simulink model "tb_mcu_rc"  (R2026b)
values from neighbouring files (symbols this model uses):
  P = evalin('base', 'P')    [elec_harness.m]    (also in mcu_can1_roundtrip.m; mcu_can2_roundtrip.m; mcu_cl_input.m; mcu_ctrl_harness.m)
  Ts = prm(1)    [mcu_cl_track_dyn.m]    (also in mcu_ctrl_harness.m = evalin('base', tsExpr))
libraries: simulink x3
settings Model: Creator=aomar  LastModifiedBy=aomar

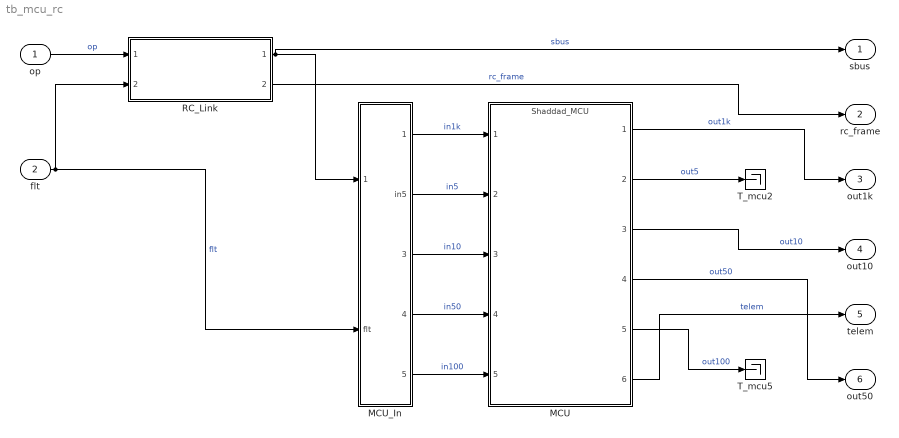
== system tb_mcu_rc ==
  op : Inport  OutDataTypeStr=Bus: Bus_OperatorCmd  SampleTime=Ts.ctrl
  flt : Inport  Port=2  OutDataTypeStr=Bus: Bus_FaultInject  SampleTime=Ts.ctrl
  MCU : ModelReference  ModelNameDialog=Shaddad_MCU  SimulationMode=Normal  ModelReferenceVersion=1.1
  MCU_In : Subsystem
  RC_Link : Subsystem  ReferencedSubsystem=RC_Link_Sim
  T_mcu2 : Terminator
  T_mcu5 : Terminator
  sbus : Outport  OutDataTypeStr=Bus: Bus_SbusStream
  rc_frame : Outport  Port=2  OutDataTypeStr=Bus: Bus_RcFrame
  out1k : Outport  Port=3  OutDataTypeStr=Bus: Bus_McuOut1k
  out10 : Outport  Port=4  OutDataTypeStr=Bus: Bus_McuOut10
  telem : Outport  Port=5  OutDataTypeStr=Bus: Bus_FwTelemetry
  out50 : Outport  Port=6  OutDataTypeStr=Bus: Bus_McuOut50
  wires:
  op/1 -> RC_Link/1  "op"
  flt/1 -> MCU_In/2(flt), RC_Link/2  "flt"
  RC_Link/1 -> MCU_In/1(sbus), sbus/1  "sbus"
  RC_Link/2 -> rc_frame/1  "rc_frame"
  MCU_In/1(in1k) -> MCU/1  "in1k"
  MCU_In/2(in5) -> MCU/2  "in5"
  MCU_In/3(in10) -> MCU/3  "in10"
  MCU_In/4(in50) -> MCU/4  "in50"
  MCU_In/5(in100) -> MCU/5  "in100"
  MCU/1 -> out1k/1  "out1k"
  MCU/2 -> T_mcu2/1  "out5"
  MCU/3 -> out10/1  "out10"
  MCU/4 -> out50/1  "out50"
  MCU/5 -> T_mcu5/1  "out100"
  MCU/6 -> telem/1  "telem"

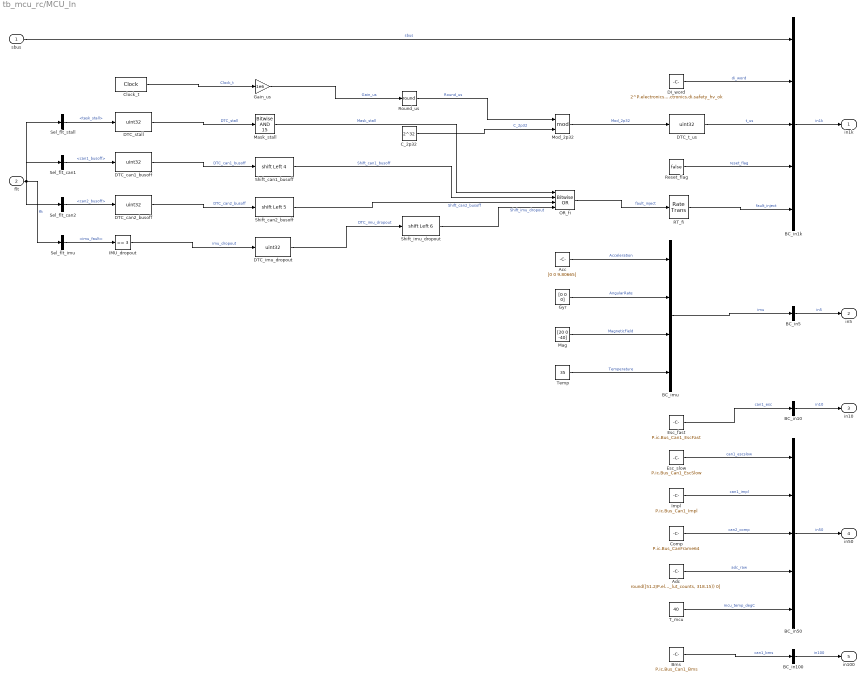
== system tb_mcu_rc/MCU_In ==
  sbus : Inport
  flt : Inport  Port=2
  Acc : Constant  Value=[0 0 9.80665]  OutDataTypeStr=single  SampleTime=Ts.imu
  Adc : Constant  Value=round([51.2/P.electronics.adc.k_vpack 51.2/P.electronics.adc.k_vlink P.electronics.adc.i_off 24/P.electronics.adc.k_v24 12/P.electronics.adc.k_v12 5/P.electronics.adc.k_v5 0 0.5*P.electronics.adc.vref]/P.electronics.adc.vref*65535) + [0 0 0 0 0 0 round(interp1(P.electronics.adc.ntc_lut_K, P.electronics.adc.ntc_lut_counts, 318.15)) 0]  OutDataTypeStr=uint16  SampleTime=Ts.comm
  BC_imu : BusCreator  Inputs=4  OutDataTypeStr=Bus: Bus_ImuRaw  NonVirtualBus=on
      settings: InheritFromInputs=off
  BC_in10 : BusCreator  Inputs=1  OutDataTypeStr=Bus: Bus_McuIn10  NonVirtualBus=on
      settings: InheritFromInputs=off
  BC_in100 : BusCreator  Inputs=1  OutDataTypeStr=Bus: Bus_McuIn100  NonVirtualBus=on
      settings: InheritFromInputs=off
  BC_in1k : BusCreator  Inputs=5  OutDataTypeStr=Bus: Bus_McuIn1k  NonVirtualBus=on
      settings: InheritFromInputs=off
  BC_in5 : BusCreator  Inputs=1  OutDataTypeStr=Bus: Bus_McuIn5  NonVirtualBus=on
      settings: InheritFromInputs=off
  BC_in50 : BusCreator  Inputs=5  OutDataTypeStr=Bus: Bus_McuIn50  NonVirtualBus=on
      settings: InheritFromInputs=off
  Bms : Constant  Value=P.ic.Bus_Can1_Bms  OutDataTypeStr=Bus: Bus_Can1_Bms  SampleTime=Ts.hk
  C_2p32 : Constant  Value=2^32  OutDataTypeStr=double  SampleTime=Ts.base
  Clock_t : DigitalClock  SampleTime=Ts.base
  Comp : Constant  Value=P.ic.Bus_CanFrame64  OutDataTypeStr=Bus: Bus_CanFrame64  SampleTime=Ts.comm
  DI_word : Constant  Value=2^P.electronics.di.estop_ch1_ok + 2^P.electronics.di.estop_ch2_ok + 2^P.electronics.di.safety_ok + 2^P.electronics.di.lid_closed + 2^P.electronics.di.key_on + 2^P.electronics.di.safety_hv_ok  OutDataTypeStr=uint16  SampleTime=Ts.base
  DTC_can1_busoff : DataTypeConversion  OutDataTypeStr=uint32  SaturateOnIntegerOverflow=off  RndMeth=Floor
  DTC_can2_busoff : DataTypeConversion  OutDataTypeStr=uint32  SaturateOnIntegerOverflow=off  RndMeth=Floor
  DTC_imu_dropout : DataTypeConversion  OutDataTypeStr=uint32  SaturateOnIntegerOverflow=off  RndMeth=Floor
  DTC_stall : DataTypeConversion  OutDataTypeStr=uint32  SaturateOnIntegerOverflow=off  RndMeth=Floor
  DTC_t_us : DataTypeConversion  OutDataTypeStr=uint32  SaturateOnIntegerOverflow=off  RndMeth=Floor
  Esc_fast : Constant  Value=P.ic.Bus_Can1_EscFast  OutDataTypeStr=Bus: Bus_Can1_EscFast  SampleTime=Ts.ctrl
  Esc_slow : Constant  Value=P.ic.Bus_Can1_EscSlow  OutDataTypeStr=Bus: Bus_Can1_EscSlow  SampleTime=Ts.comm
  Gain_us : Gain  Gain=1e6
  Gyr : Constant  Value=[0 0 0]  OutDataTypeStr=single  SampleTime=Ts.imu
  IMU_dropout : simulink/Logic and Bit Operations/Compare To Constant  relop===  const=3  OutDataTypeStr=boolean
  Impl : Constant  Value=P.ic.Bus_Can1_Impl  OutDataTypeStr=Bus: Bus_Can1_Impl  SampleTime=Ts.comm
  Mag : Constant  Value=[20 0 -40]  OutDataTypeStr=single  SampleTime=Ts.imu
  Mask_stall : simulink/Logic and Bit Operations/Bitwise Operator  logicop=AND  UseBitMask=on  BitMask=15  BitMaskRealWorld=Stored Integer
  Mod_2p32 : Math  Operator=mod
  OR_fi : simulink/Logic and Bit Operations/Bitwise Operator  logicop=OR  UseBitMask=off  NumInputPorts=4  BitMask=bin2dec('11011001')  BitMaskRealWorld=Stored Integer
  RT_fi : RateTransition  OutPortSampleTime=Ts.base
  Reset_flag : Constant  Value=false  OutDataTypeStr=boolean  SampleTime=Ts.base
  Round_us : Rounding  Operator=round
  Sel_flt_can1 : BusSelector  OutputSignals=can1_busoff
  Sel_flt_can2 : BusSelector  OutputSignals=can2_busoff
  Sel_flt_imu : BusSelector  OutputSignals=imu_fault
  Sel_flt_stall : BusSelector  OutputSignals=task_stall
  Shift_can1_busoff : ArithShift  BitShiftNumber=4  BitShiftDirection=Left
  Shift_can2_busoff : ArithShift  BitShiftNumber=5  BitShiftDirection=Left
  Shift_imu_dropout : ArithShift  BitShiftNumber=6  BitShiftDirection=Left
  T_mcu : Constant  Value=40  OutDataTypeStr=single  SampleTime=Ts.comm
  Temp : Constant  Value=35  OutDataTypeStr=single  SampleTime=Ts.imu
  in1k : Outport
  in5 : Outport  Port=2
  in10 : Outport  Port=3
  in50 : Outport  Port=4
  in100 : Outport  Port=5
  wires:
  sbus/1 -> BC_in1k/1  "sbus"
  flt/1 -> Sel_flt_imu/1, Sel_flt_stall/1, Sel_flt_can2/1, Sel_flt_can1/1  "flt"
  Sel_flt_stall/1 -> DTC_stall/1  "<task_stall>"
  Sel_flt_can1/1 -> DTC_can1_busoff/1  "<can1_busoff>"
  Sel_flt_can2/1 -> DTC_can2_busoff/1  "<can2_busoff>"
  Sel_flt_imu/1 -> IMU_dropout/1  "<imu_fault>"
  IMU_dropout/1 -> DTC_imu_dropout/1  "imu_dropout"
  Clock_t/1 -> Gain_us/1  "Clock_t"
  DTC_stall/1 -> Mask_stall/1  "DTC_stall"
  DTC_can1_busoff/1 -> Shift_can1_busoff/1  "DTC_can1_busoff"
  DTC_can2_busoff/1 -> Shift_can2_busoff/1  "DTC_can2_busoff"
  Gain_us/1 -> Round_us/1  "Gain_us"
  Mask_stall/1 -> OR_fi/1  "Mask_stall"
  DTC_imu_dropout/1 -> Shift_imu_dropout/1  "DTC_imu_dropout"
  Shift_can1_busoff/1 -> OR_fi/2  "Shift_can1_busoff"
  Shift_can2_busoff/1 -> OR_fi/3  "Shift_can2_busoff"
  Round_us/1 -> Mod_2p32/1  "Round_us"
  C_2p32/1 -> Mod_2p32/2  "C_2p32"
  Shift_imu_dropout/1 -> OR_fi/4  "Shift_imu_dropout"
  Mod_2p32/1 -> DTC_t_us/1  "Mod_2p32"
  Acc/1 -> BC_imu/1  "Acceleration"
  Gyr/1 -> BC_imu/2  "AngularRate"
  Mag/1 -> BC_imu/3  "MagneticField"
  Temp/1 -> BC_imu/4  "Temperature"
  OR_fi/1 -> RT_fi/1  "fault_inject"
  BC_imu/1 -> BC_in5/1  "imu"
  DI_word/1 -> BC_in1k/2  "di_word"
  Reset_flag/1 -> BC_in1k/4  "reset_flag"
  Esc_fast/1 -> BC_in10/1  "can1_esc"
  Esc_slow/1 -> BC_in50/1  "can1_escslow"
  Impl/1 -> BC_in50/2  "can1_impl"
  Comp/1 -> BC_in50/3  "can2_comp"
  Adc/1 -> BC_in50/4  "adc_raw"
  T_mcu/1 -> BC_in50/5  "mcu_temp_degC"
  Bms/1 -> BC_in100/1  "can1_bms"
  RT_fi/1 -> BC_in1k/5  "fault_inject"
  DTC_t_us/1 -> BC_in1k/3  "t_us"
  BC_in1k/1 -> in1k/1  "in1k"
  BC_in5/1 -> in5/1  "in5"
  BC_in10/1 -> in10/1  "in10"
  BC_in50/1 -> in50/1  "in50"
  BC_in100/1 -> in100/1  "in100"
